simulink model "ares_single_uav_top_dirty_backup_20261011"  (R2026a)
settings: Solver=VariableStepAuto  StopTime=60
undefined symbols (not defined in the file or in its folder): DroneMass, Dx, Dy, Dz, Gravity, Ix, Iy, Iz, Lidar, MaxRange, Nx, Ny, Nz, Px, Py, Pz, UAV, Waypoints
libraries: slpidlib x6, uavsimlib x5, uavalgslib x3, robotcorelib x2
settings Model: NumberOfSteps=100  PacingRate=10  Creator=The MathWorks, Inc.  LastModifiedBy=athar
settings DebuggingCC: ParameterPrecisionLossMsg=none

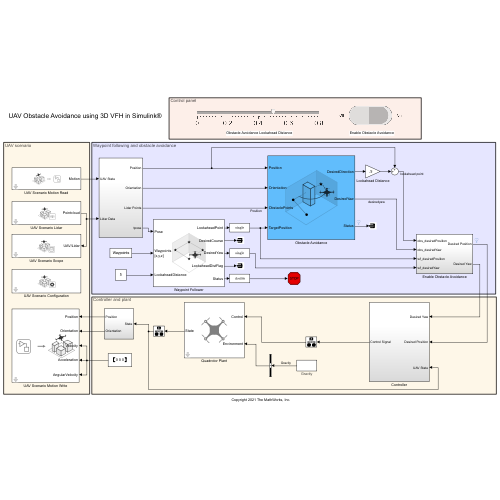
[thumbnail: Simulink's stored preview of the top-level diagram]
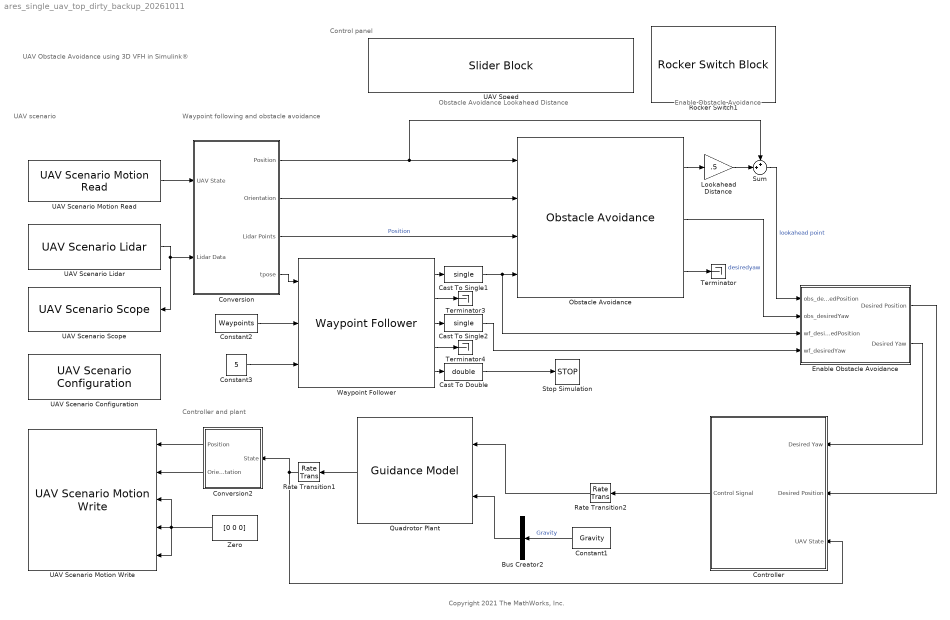
== system ares_single_uav_top_dirty_backup_20261011 ==
  note: Copyright 2021 The MathWorks, Inc.
  note: Control panel
  note: Enable Obstacle Avoidance
  note: Obstacle Avoidance Lookahead Distance
  note: Waypoint following and obstacle avoidance
  note: UAV scenario
  note: Controller and plant
  note: UAV Obstacle Avoidance using 3D VFH in Simulink®
  Bus Creator2 : BusCreator  Inputs=1  OutDataTypeStr=Bus: uavGuidanceEnvironmentBus  NonVirtualBus=on
  Cast To Double : DataTypeConversion  OutDataTypeStr=double  SaturateOnIntegerOverflow=off  RndMeth=Floor
  Cast To Single1 : DataTypeConversion  OutDataTypeStr=single  SaturateOnIntegerOverflow=off  RndMeth=Floor
  Cast To Single2 : DataTypeConversion  OutDataTypeStr=single  SaturateOnIntegerOverflow=off  RndMeth=Floor
  Constant1 : Constant  Value=Gravity  OutDataTypeStr=single
      settings: AttributesFormatString=%<Value>
  Constant2 : Constant  Value=Waypoints
  Constant3 : Constant  Value=5
  Controller : Subsystem
  Conversion : Subsystem
  Conversion2 : Subsystem
  Enable Obstacle Avoidance : Subsystem
  Lookahead Distance : Gain  Gain=.5
  Obstacle Avoidance : uavalgslib/Obstacle Avoidance  DistanceLimits=[ 0.2, MaxRange]  HorizontalSensorFOV=AzimuthLimits  VerticalSensorFOV=ElevationLimits  SensorLocation=[ 0, 0, -0.4]  SensorOrientation=[ 180, 0, 0 ]  VehicleRadius=VehicleRadius  SafetyDistance=AvoidanceSafetyDistance  SimulateUsing=Interpreted execution  HistRes=6  WindowSize=1  HistogramThreshold=1  MaxAge=3  TargetDirectionWeight=5  CurrentDirectionWeight=2  PreviousDirectionWeight=2
  Quadrotor Plant : uavalgslib/Guidance Model  ModelType=MultirotorGuidance  NumInstances=1  SpecifiedDataType=single  SimulateUsing=Code generation  InitialWorldPositionMultirotor=InitialPosition'  InitialWorldVelocityMultirotor=[0; 0; 0]  InitialEulerZYXMultirotor=|  InitialBodyAngularRateRPYMultirotor=[0; 0; 0]  InitialThrustMultirotor=0  InitialNorthFixedWing=0  InitialEastFixedWing=0  InitialHeightFixedWing=0  InitialAirSpeedFixedWing=0  InitialHeadingAngleFixedWing=0  InitialFlightPathAngleFixedWing=0  InitialRollAngleFixedWing=0  InitialRollAngleRateFixedWing=0  PDRollMultirotor=[3402.97,116.67]  PDPitchMultirotor=[3402.97, 116.67]  PYawRateMultirotor=1950  PThrustMultirotor=3900  MassMultirotor=0.1  PHeightFixedWing=3.9  PHeadingAngleFixedWing=3.9  PFlightPathAngleFixedWing=39  PDRollFixedWing=[3402.97, 116.67]  PAirSpeedFixedWing=1  FlightPathAngleLimitsFixedWing=[-pi/2, pi/2]  StateBusName='uavGuidanceStateBus'  ControlBusName='uavGuidanceControlBus'  EnvironmentBusName='uavGuidanceEnvironmentBus'  DataType=single
      | [ 0
      | ;0;0]
      link override EnvironmentSignalSpecification: OutDataTypeStr=Bus: MultirotorGuidanceEnvironmentBus
  Rate Transition1 : RateTransition  OutPortSampleTime=UAVSampleTime
  Rate Transition2 : RateTransition  OutPortSampleTime=UAVSampleTime
  Rocker Switch1 : RockerSwitchBlock  LabelPosition=Hide
  Stop Simulation : Stop
  Sum : Sum  Inputs=++|
  Terminator : Terminator
  Terminator3 : Terminator
  Terminator4 : Terminator
  UAV Scenario Configuration : uavsimlib/UAV Scenario Configuration  Priority=-1  UAVScenarioObject=Scenario  SampleTime=0.1  UpdateParam=true  SensorMotionBusName='SensorMotionBus'  PlatformMotionBusName='PlatformMotionBus'  ScenarioMotionBusName='ScenarioMotionBus'  ScenarioMotionSignalName='ScenarioMotions'
  UAV Scenario Lidar : uavsimlib/UAV Scenario Lidar  Priority=1  SensorName=UAV/Lidar  MaxRange=MaxRange  RangeAccuracy=0.02  AzimuthLimits=AzimuthLimits  AzimuthResolution=AzimuthResolution  ElevationLimits=ElevationLimits  ElevationResolution=ElevationResolution  HasNoise=off  HasOrganizedOutput=on  SampleTime=0.1
  UAV Scenario Motion Read : uavsimlib/UAV Scenario Motion Read  Priority=1  EntityName='UAV'  ReferenceFrame=NED  OutputWind=off
  UAV Scenario Motion Write : uavsimlib/UAV Scenario Motion Write  Priority=0  PlatName='UAV'  ReferenceFrame=NED
  UAV Scenario Scope : uavsimlib/UAV Scenario Scope  Priority=1  SensorNameTable={ 'UAV/Lidar', 'on' }  SampleTime=.1
  UAV Speed : SliderBlock  LabelPosition=Hide  ScaleMin=0.0  ScaleMax=.8  TickInterval=.2
  Waypoint Follower : uavalgslib/Waypoint Follower  UAVType=multirotor  StartFrom=first  TransitionRadiusSource=internal  TransitionRadius=.1  MinLookaheadDistance=.2  HoverAtLastWaypoint=off  InterpolateYaw=on  YawInput=off  ShowCrossTrackErrorOutput=off  ShowStatusOutput=on  ShowWaypointIndexOutput=off  SimulateUsing=Code generation
  Zero : Constant  Value=[0 0 0]  OutDataTypeStr=Inherit: Inherit via back propagation
  wires:
  Controller/1(Control Signal) -> Rate Transition2/1
  Rate Transition2/1 -> Quadrotor Plant/1
  Obstacle Avoidance/1 -> Lookahead Distance/1
  Rate Transition1/1 -> Controller/3(UAV State), Conversion2/1(State)
  Quadrotor Plant/1 -> Rate Transition1/1
  Conversion/1(Position) -> Sum/1, Obstacle Avoidance/1
  Conversion/2(Orientation) -> Obstacle Avoidance/2
  Bus Creator2/1 -> Quadrotor Plant/2
  Constant1/1 -> Bus Creator2/1  "Gravity"
  Lookahead Distance/1 -> Sum/2
  Obstacle Avoidance/3 -> Terminator/1
  Conversion/3(Lidar Points) -> Obstacle Avoidance/3  "Position"
  UAV Scenario Motion Read/1 -> Conversion/1(UAV State)
  UAV Scenario Lidar/1 -> UAV Scenario Scope/1, Conversion/2(Lidar Data)
  Conversion2/1(Position) -> UAV Scenario Motion Write/1
  Conversion2/2(Orientation) -> UAV Scenario Motion Write/2
  Zero/1 -> UAV Scenario Motion Write/3, UAV Scenario Motion Write/4, UAV Scenario Motion Write/5
  Waypoint Follower/5 -> Cast To Double/1
  Waypoint Follower/4 -> Terminator4/1
  Waypoint Follower/2 -> Terminator3/1
  Constant3/1 -> Waypoint Follower/3
  Waypoint Follower/1 -> Cast To Single1/1
  Constant2/1 -> Waypoint Follower/2
  Conversion/4(tpose) -> Waypoint Follower/1
  Cast To Single1/1 -> Enable Obstacle Avoidance/3(wf_desiredPosition), Obstacle Avoidance/4
  Cast To Double/1 -> Stop Simulation/1
  Waypoint Follower/3 -> Cast To Single2/1
  Sum/1 -> Enable Obstacle Avoidance/1(obs_desiredPosition)  "lookahead point"
  Obstacle Avoidance/2 -> Enable Obstacle Avoidance/2(obs_desiredYaw)  "desiredyaw"
  Cast To Single2/1 -> Enable Obstacle Avoidance/4(wf_desiredYaw)
  Enable Obstacle Avoidance/2(Desired Yaw) -> Controller/1(Desired Yaw)
  Enable Obstacle Avoidance/1(Desired Position) -> Controller/2(Desired Position)

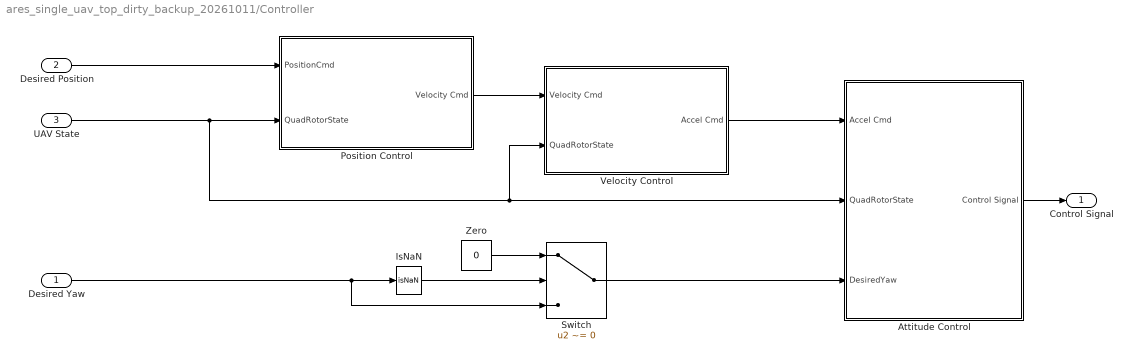
== system ares_single_uav_top_dirty_backup_20261011/Controller ==
  Desired Yaw : Inport
  Desired Position : Inport  Port=2
  UAV State : Inport  Port=3
  Attitude Control : Subsystem
  IsNaN : RelationalOperator  Operator=isNaN  OutDataTypeStr=boolean  RndMeth=Simplest  InputSameDT=off
  Position Control : Subsystem
  Switch : Switch  Criteria=u2 ~= 0  SaturateOnIntegerOverflow=off  InputSameDT=off
  Velocity Control : Subsystem
  Zero : Constant  Value=0  OutDataTypeStr=Inherit: Inherit via back propagation
  Control Signal : Outport
  wires:
  Desired Position/1 -> Position Control/1(PositionCmd)
  Velocity Control/1(Accel Cmd) -> Attitude Control/1(Accel Cmd)
  Attitude Control/1(Control Signal) -> Control Signal/1
  UAV State/1 -> Position Control/2(QuadRotorState), Velocity Control/2(QuadRotorState), Attitude Control/2(QuadRotorState)
  Position Control/1(Velocity Cmd) -> Velocity Control/1(Velocity Cmd)
  Zero/1 -> Switch/1
  IsNaN/1 -> Switch/2
  Desired Yaw/1 -> Switch/3, IsNaN/1
  Switch/1 -> Attitude Control/3(DesiredYaw)

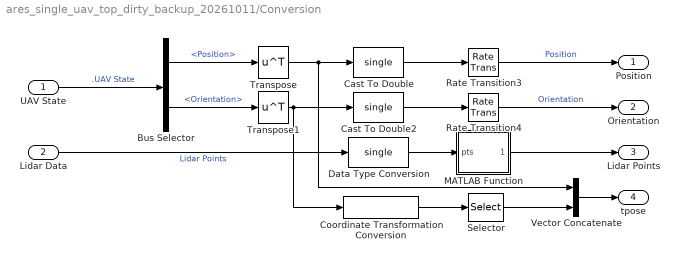
== system ares_single_uav_top_dirty_backup_20261011/Conversion ==
  UAV State : Inport
  Lidar Data : Inport  Port=2
  Bus Selector : BusSelector  OutputSignals=Position,Orientation
  Cast To Double : DataTypeConversion  OutDataTypeStr=single  SaturateOnIntegerOverflow=off  RndMeth=Floor
  Cast To Double2 : DataTypeConversion  OutDataTypeStr=single  SaturateOnIntegerOverflow=off  RndMeth=Floor
  Coordinate Transformation Conversion : robotcorelib/Coordinate Transformation Conversion  InputRepresentation=Quaternion  InputEulerSequence=ZYX  ShowTrVecInputPort=on  OutputRepresentation=Euler Angles  OutputEulerSequence=ZYX  ShowTrVecOutputPort=on  SimulateUsing=Interpreted execution
  Data Type Conversion : DataTypeConversion  OutDataTypeStr=single  SaturateOnIntegerOverflow=off  RndMeth=Floor
  MATLAB Function : MATLAB Function  TreatAsAtomicUnit=on
  Rate Transition3 : RateTransition  OutPortSampleTime=.1
  Rate Transition4 : RateTransition  OutPortSampleTime=0.1
  Selector : Selector  InputPortWidth=3  IndexOptions=Index vector (dialog)  Indices=[1]  OutputSizes=1
  Transpose : Math  Operator=transpose
  Transpose1 : Math  Operator=transpose
  Vector Concatenate : Concatenate
  Position : Outport
  Orientation : Outport  Port=2
  Lidar Points : Outport  Port=3
  tpose : Outport  Port=4
  wires:
  Bus Selector/2 -> Transpose1/1  "<Orientation>"
  Data Type Conversion/1 -> MATLAB Function/1(pts)
  Bus Selector/1 -> Transpose/1  "<Position>"
  Transpose1/1 -> Coordinate Transformation Conversion/1, Cast To Double2/1
  Transpose/1 -> Cast To Double/1, Vector Concatenate/1
  Cast To Double2/1 -> Rate Transition4/1
  UAV State/1 -> Bus Selector/1  ".UAV State"
  Lidar Data/1 -> Data Type Conversion/1  "Lidar Points"
  Rate Transition4/1 -> Orientation/1  "Orientation"
  MATLAB Function/1(points) -> Lidar Points/1
  Rate Transition3/1 -> Position/1  "Position"
  Vector Concatenate/1 -> tpose/1
  Selector/1 -> Vector Concatenate/2
  Cast To Double/1 -> Rate Transition3/1
  Coordinate Transformation Conversion/1 -> Selector/1

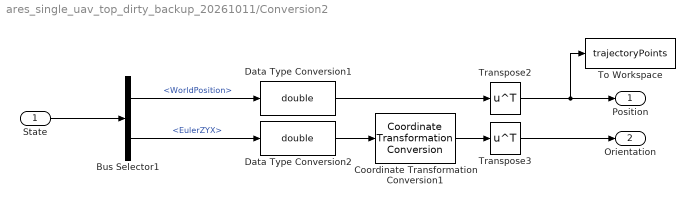
== system ares_single_uav_top_dirty_backup_20261011/Conversion2 ==
  State : Inport
  Bus Selector1 : BusSelector  OutputSignals=WorldPosition,EulerZYX
  Coordinate Transformation Conversion1 : robotcorelib/Coordinate Transformation Conversion  InputRepresentation=Euler Angles  InputEulerSequence=ZYX  ShowTrVecInputPort=on  OutputRepresentation=Quaternion  OutputEulerSequence=ZYX  ShowTrVecOutputPort=on  SimulateUsing=Code generation
  Data Type Conversion1 : DataTypeConversion  OutDataTypeStr=double  SaturateOnIntegerOverflow=off  RndMeth=Floor
  Data Type Conversion2 : DataTypeConversion  OutDataTypeStr=double  SaturateOnIntegerOverflow=off  RndMeth=Floor
  To Workspace : ToWorkspace  VariableName=trajectoryPoints  SampleTime=-1
  Transpose2 : Math  Operator=transpose
  Transpose3 : Math  Operator=transpose
  Position : Outport
  Orientation : Outport  Port=2
  wires:
  State/1 -> Bus Selector1/1
  Transpose2/1 -> To Workspace/1, Position/1
  Bus Selector1/1 -> Data Type Conversion1/1  "<WorldPosition>"
  Data Type Conversion2/1 -> Coordinate Transformation Conversion1/1
  Bus Selector1/2 -> Data Type Conversion2/1  "<EulerZYX>"
  Coordinate Transformation Conversion1/1 -> Transpose3/1
  Transpose3/1 -> Orientation/1
  Data Type Conversion1/1 -> Transpose2/1

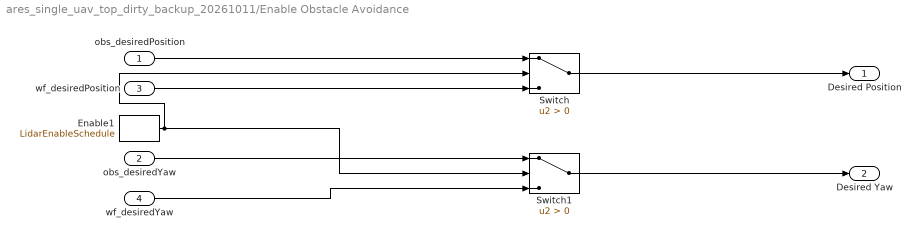
== system ares_single_uav_top_dirty_backup_20261011/Enable Obstacle Avoidance ==
  obs_desiredPosition : Inport
  obs_desiredYaw : Inport  Port=2
  wf_desiredPosition : Inport  Port=3
  wf_desiredYaw : Inport  Port=4
  Enable1 : FromWorkspace  VariableName=LidarEnableSchedule  Interpolate=off  OutputAfterFinalValue=Holding final value
  Switch : Switch  Criteria=u2 > Threshold  SaturateOnIntegerOverflow=off  InputSameDT=off
  Switch1 : Switch  Criteria=u2 > Threshold  SaturateOnIntegerOverflow=off  InputSameDT=off
  Desired Position : Outport
  Desired Yaw : Outport  Port=2
  wires:
  wf_desiredYaw/1 -> Switch1/3
  obs_desiredYaw/1 -> Switch1/1
  Switch/1 -> Desired Position/1
  obs_desiredPosition/1 -> Switch/1
  Switch1/1 -> Desired Yaw/1
  wf_desiredPosition/1 -> Switch/3
  Enable1/1 -> Switch/2, Switch1/2

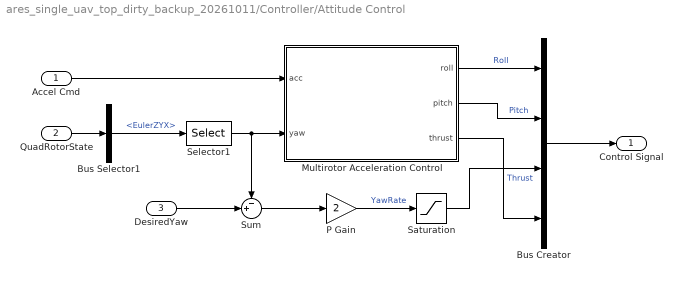
== system ares_single_uav_top_dirty_backup_20261011/Controller/Attitude Control ==
  Accel Cmd : Inport
  QuadRotorState : Inport  Port=2
  DesiredYaw : Inport  Port=3
  Bus Creator : BusCreator  Inputs=4  OutDataTypeStr=Bus: uavGuidanceControlBus  NonVirtualBus=on
      settings: InheritFromInputs=off
  Bus Selector1 : BusSelector  OutputSignals=EulerZYX
  Multirotor Acceleration Control : MATLAB Function  TreatAsAtomicUnit=on
  P Gain : Gain  Gain=2
  Saturation : Saturate
  Selector1 : Selector  InputPortWidth=3  IndexOptions=Index vector (dialog)  Indices=[1]  OutputSizes=1
  Sum : Sum  Inputs=-+|
  Control Signal : Outport
  wires:
  Selector1/1 -> Multirotor Acceleration Control/2(yaw), Sum/1
  Bus Creator/1 -> Control Signal/1
  Sum/1 -> P Gain/1
  Multirotor Acceleration Control/1(roll) -> Bus Creator/1  "Roll"
  Multirotor Acceleration Control/2(pitch) -> Bus Creator/2  "Pitch"
  Multirotor Acceleration Control/3(thrust) -> Bus Creator/4  "Thrust"
  P Gain/1 -> Saturation/1  "YawRate"
  Accel Cmd/1 -> Multirotor Acceleration Control/1(acc)
  QuadRotorState/1 -> Bus Selector1/1
  Bus Selector1/1 -> Selector1/1  "<EulerZYX>"
  Saturation/1 -> Bus Creator/3
  DesiredYaw/1 -> Sum/2

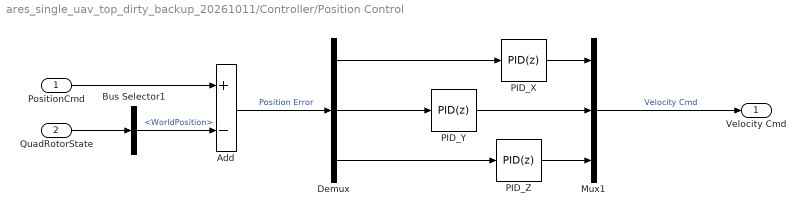
== system ares_single_uav_top_dirty_backup_20261011/Controller/Position Control ==
  PositionCmd : Inport
  QuadRotorState : Inport  Port=2
  Add : Sum  Inputs=+-
  Bus Selector1 : BusSelector  OutputSignals=WorldPosition
  Demux : Demux  Outputs=3
  Mux1 : Mux  Inputs=3
  PID_X : slpidlib/PID Controller  Controller=PID  Form=Parallel  TimeDomain=Discrete-time  UseExternalTs=off  SampleTime=-1  IntegratorMethod=Forward Euler  FilterMethod=Forward Euler  ControllerParametersSource=internal  P=Px  I=Ix  UseKiTs=off  D=Dx  UseExternalDerivativeSource=off  N=Nx  UseFilter=on  TunerSelectOption=Transfer Function Based (PID Tuner App)  InitialConditionSource=internal  InitialConditionForIntegrator=0  InitialConditionForFilter=0  DifferentiatorICPrevScaledInput=0  ExternalReset=none  TrackingMode=off  Kt=1  LimitOutput=on  SatLimitsSource=internal  UpperSaturationLimit=3  LowerSaturationLimit=-3  LinearizeAsGain=on  AntiWindupMode=clamping  Kb=1  LimitIntegrator=off  UpperIntegratorSaturationLimit=inf  LowerIntegratorSaturationLimit=-inf  POutMin=[]  POutMax=[]  IOutMin=[]  IOutMax=[]  DOutMin=[]  DOutMax=[]  NOutMin=[]  NOutMax=[]  SumOutMin=[]  SumOutMax=[]  SaturationOutMin=[]  SaturationOutMax=[]  PParamMin=[]  PParamMax=[]  IParamMin=[]  IParamMax=[]  DParamMin=[]  DParamMax=[]  NParamMin=[]  NParamMax=[]  KbParamMin=[]  KbParamMax=[]  KtParamMin=[]  KtParamMax=[]  KbOutMin=[]  KbOutMax=[]  KtOutMin=[]  KtOutMax=[]  IntegratorOutMin=[]  IntegratorOutMax=[]  FilterOutMin=[]  FilterOutMax=[]  SumI1OutMin=SumI1OutMin  SumI1OutMax=SumI1OutMax  SumI2OutMin=[]  SumI2OutMax=[]  SumI3OutMin=[]  SumI3OutMax=[]  SumI4OutMin=[]  SumI4OutMax=[]  SumDOutMin=[]  SumDOutMax=[]  DifferentiatorOutMin=[]  DifferentiatorOutMax=[]  FilterDiffOutCoefMin=[]  FilterDiffOutCoefMax=[]  ReciprocalOutMin=[]  ReciprocalOutMax=[]  SumDenOutMin=[]  SumDenOutMax=[]  SumNumOutMin=[]  SumNumOutMax=[]  DivideOutMin=[]  DivideOutMax=[]  UdiffTsProdOutMin=[]  UdiffTsProdOutMax=[]  NTsProdOutMin=[]  NTsProdOutMax=[]  UintegralTsProdOutMin=[]  UintegralTsProdOutMax=[]  UngainTsProdOutMin=[]  UngainTsProdOutMax=[]  ClampingZeroOutDataTypeStr=Inherit: Inherit via back propagation  ClampingZeroOutMin=[]  ClampingZeroOutMax=[]  FilterDenConstantOutDataTypeStr=Inherit: Inherit via back propagation  FilterDenConstantOutMin=[]  FilterDenConstantOutMax=[]  PCopyOutDataTypeStr=Inherit: Inherit via back propagation  PCopyOutMin=[]  PCopyOutMax=[]  NCopyOutDataTypeStr=Inherit: Inherit via back propagation  NCopyOutMin=[]  NCopyOutMax=[]  IntegratorContinuousStateAttributes=''  IntegratorStateMustResolveToSignalObject=off  IntegratorRTWStateStorageClass=Auto  FilterContinuousStateAttributes=''  FilterStateMustResolveToSignalObject=off  FilterRTWStateStorageClass=Auto  ParallelPVariant=InternalParameters  IdealPVariant=Disabled  IVariant=InternalParameters  DVariant=InternalParameters  IntegratorVariant=Discrete  SatVariant=Enabled  AWVariant=DiscClampingParallel  PCopyVariant=Disabled  TRVariant=Disabled  FdbkBlocksVariant=Forward  IdealPFdbkVariant=Disabled  SatFdbkVariant=Disabled  DerivativeFilterVariant=ForwardEulerFilter  NVariant=InternalParameters  NCopyVariant=Disabled  FilterICVariant=InternalICsFilter  IntegratorICVariant=InternalICs  ExternalResetVariant=Disabled  TRSumVariant=Passthrough  SumFdbkVariant=Disabled  SumVariant=Sum_PID  TsampFilterVariant=InternalTs  TsampNgainVariant=Passthrough  TsampIntegralVariant=Disabled_SignalSpec  ExternalSaturationOutDataTypeStr=Inherit: Same as second input  DerivativeSourceVariant=ErrorSignal  PreIntVariant=InternalPreInt
      settings: AttributesFormatString=P: %<P>, I: %<I>, D:%<D>
  PID_Y : slpidlib/PID Controller  Controller=PID  Form=Parallel  TimeDomain=Discrete-time  UseExternalTs=off  SampleTime=-1  IntegratorMethod=Forward Euler  FilterMethod=Forward Euler  ControllerParametersSource=internal  P=Py  I=Iy  UseKiTs=off  D=Dy  UseExternalDerivativeSource=off  N=Ny  UseFilter=on  TunerSelectOption=Transfer Function Based (PID Tuner App)  InitialConditionSource=internal  InitialConditionForIntegrator=0  InitialConditionForFilter=0  DifferentiatorICPrevScaledInput=0  ExternalReset=none  TrackingMode=off  Kt=1  LimitOutput=on  SatLimitsSource=internal  UpperSaturationLimit=3  LowerSaturationLimit=-3  LinearizeAsGain=on  AntiWindupMode=clamping  Kb=1  LimitIntegrator=off  UpperIntegratorSaturationLimit=inf  LowerIntegratorSaturationLimit=-inf  POutMin=[]  POutMax=[]  IOutMin=[]  IOutMax=[]  DOutMin=[]  DOutMax=[]  NOutMin=[]  NOutMax=[]  SumOutMin=[]  SumOutMax=[]  SaturationOutMin=[]  SaturationOutMax=[]  PParamMin=[]  PParamMax=[]  IParamMin=[]  IParamMax=[]  DParamMin=[]  DParamMax=[]  NParamMin=[]  NParamMax=[]  KbParamMin=[]  KbParamMax=[]  KtParamMin=[]  KtParamMax=[]  KbOutMin=[]  KbOutMax=[]  KtOutMin=[]  KtOutMax=[]  IntegratorOutMin=[]  IntegratorOutMax=[]  FilterOutMin=[]  FilterOutMax=[]  SumI1OutMin=SumI1OutMin  SumI1OutMax=SumI1OutMax  SumI2OutMin=[]  SumI2OutMax=[]  SumI3OutMin=[]  SumI3OutMax=[]  SumI4OutMin=[]  SumI4OutMax=[]  SumDOutMin=[]  SumDOutMax=[]  DifferentiatorOutMin=[]  DifferentiatorOutMax=[]  FilterDiffOutCoefMin=[]  FilterDiffOutCoefMax=[]  ReciprocalOutMin=[]  ReciprocalOutMax=[]  SumDenOutMin=[]  SumDenOutMax=[]  SumNumOutMin=[]  SumNumOutMax=[]  DivideOutMin=[]  DivideOutMax=[]  UdiffTsProdOutMin=[]  UdiffTsProdOutMax=[]  NTsProdOutMin=[]  NTsProdOutMax=[]  UintegralTsProdOutMin=[]  UintegralTsProdOutMax=[]  UngainTsProdOutMin=[]  UngainTsProdOutMax=[]  ClampingZeroOutDataTypeStr=Inherit: Inherit via back propagation  ClampingZeroOutMin=[]  ClampingZeroOutMax=[]  FilterDenConstantOutDataTypeStr=Inherit: Inherit via back propagation  FilterDenConstantOutMin=[]  FilterDenConstantOutMax=[]  PCopyOutDataTypeStr=Inherit: Inherit via back propagation  PCopyOutMin=[]  PCopyOutMax=[]  NCopyOutDataTypeStr=Inherit: Inherit via back propagation  NCopyOutMin=[]  NCopyOutMax=[]  IntegratorContinuousStateAttributes=''  IntegratorStateMustResolveToSignalObject=off  IntegratorRTWStateStorageClass=Auto  FilterContinuousStateAttributes=''  FilterStateMustResolveToSignalObject=off  FilterRTWStateStorageClass=Auto  ParallelPVariant=InternalParameters  IdealPVariant=Disabled  IVariant=InternalParameters  DVariant=InternalParameters  IntegratorVariant=Discrete  SatVariant=Enabled  AWVariant=DiscClampingParallel  PCopyVariant=Disabled  TRVariant=Disabled  FdbkBlocksVariant=Forward  IdealPFdbkVariant=Disabled  SatFdbkVariant=Disabled  DerivativeFilterVariant=ForwardEulerFilter  NVariant=InternalParameters  NCopyVariant=Disabled  FilterICVariant=InternalICsFilter  IntegratorICVariant=InternalICs  ExternalResetVariant=Disabled  TRSumVariant=Passthrough  SumFdbkVariant=Disabled  SumVariant=Sum_PID  TsampFilterVariant=InternalTs  TsampNgainVariant=Passthrough  TsampIntegralVariant=Disabled_SignalSpec  ExternalSaturationOutDataTypeStr=Inherit: Same as second input  DerivativeSourceVariant=ErrorSignal  PreIntVariant=InternalPreInt
      settings: AttributesFormatString=P: %<P>, I: %<I>, D:%<D>
  PID_Z : slpidlib/PID Controller  Controller=PID  Form=Parallel  TimeDomain=Discrete-time  UseExternalTs=off  SampleTime=-1  IntegratorMethod=Forward Euler  FilterMethod=Forward Euler  ControllerParametersSource=internal  P=Pz  I=Iz  UseKiTs=off  D=Dz  UseExternalDerivativeSource=off  N=Nz  UseFilter=on  TunerSelectOption=Transfer Function Based (PID Tuner App)  InitialConditionSource=internal  InitialConditionForIntegrator=0  InitialConditionForFilter=0  DifferentiatorICPrevScaledInput=0  ExternalReset=none  TrackingMode=off  Kt=1  LimitOutput=on  SatLimitsSource=internal  UpperSaturationLimit=3  LowerSaturationLimit=-3  LinearizeAsGain=on  AntiWindupMode=clamping  Kb=1  LimitIntegrator=off  UpperIntegratorSaturationLimit=inf  LowerIntegratorSaturationLimit=-inf  POutMin=[]  POutMax=[]  IOutMin=[]  IOutMax=[]  DOutMin=[]  DOutMax=[]  NOutMin=[]  NOutMax=[]  SumOutMin=[]  SumOutMax=[]  SaturationOutMin=[]  SaturationOutMax=[]  PParamMin=[]  PParamMax=[]  IParamMin=[]  IParamMax=[]  DParamMin=[]  DParamMax=[]  NParamMin=[]  NParamMax=[]  KbParamMin=[]  KbParamMax=[]  KtParamMin=[]  KtParamMax=[]  KbOutMin=[]  KbOutMax=[]  KtOutMin=[]  KtOutMax=[]  IntegratorOutMin=[]  IntegratorOutMax=[]  FilterOutMin=[]  FilterOutMax=[]  SumI1OutMin=SumI1OutMin  SumI1OutMax=SumI1OutMax  SumI2OutMin=[]  SumI2OutMax=[]  SumI3OutMin=[]  SumI3OutMax=[]  SumI4OutMin=[]  SumI4OutMax=[]  SumDOutMin=[]  SumDOutMax=[]  DifferentiatorOutMin=[]  DifferentiatorOutMax=[]  FilterDiffOutCoefMin=[]  FilterDiffOutCoefMax=[]  ReciprocalOutMin=[]  ReciprocalOutMax=[]  SumDenOutMin=[]  SumDenOutMax=[]  SumNumOutMin=[]  SumNumOutMax=[]  DivideOutMin=[]  DivideOutMax=[]  UdiffTsProdOutMin=[]  UdiffTsProdOutMax=[]  NTsProdOutMin=[]  NTsProdOutMax=[]  UintegralTsProdOutMin=[]  UintegralTsProdOutMax=[]  UngainTsProdOutMin=[]  UngainTsProdOutMax=[]  ClampingZeroOutDataTypeStr=Inherit: Inherit via back propagation  ClampingZeroOutMin=[]  ClampingZeroOutMax=[]  FilterDenConstantOutDataTypeStr=Inherit: Inherit via back propagation  FilterDenConstantOutMin=[]  FilterDenConstantOutMax=[]  PCopyOutDataTypeStr=Inherit: Inherit via back propagation  PCopyOutMin=[]  PCopyOutMax=[]  NCopyOutDataTypeStr=Inherit: Inherit via back propagation  NCopyOutMin=[]  NCopyOutMax=[]  IntegratorContinuousStateAttributes=''  IntegratorStateMustResolveToSignalObject=off  IntegratorRTWStateStorageClass=Auto  FilterContinuousStateAttributes=''  FilterStateMustResolveToSignalObject=off  FilterRTWStateStorageClass=Auto  ParallelPVariant=InternalParameters  IdealPVariant=Disabled  IVariant=InternalParameters  DVariant=InternalParameters  IntegratorVariant=Discrete  SatVariant=Enabled  AWVariant=DiscClampingParallel  PCopyVariant=Disabled  TRVariant=Disabled  FdbkBlocksVariant=Forward  IdealPFdbkVariant=Disabled  SatFdbkVariant=Disabled  DerivativeFilterVariant=ForwardEulerFilter  NVariant=InternalParameters  NCopyVariant=Disabled  FilterICVariant=InternalICsFilter  IntegratorICVariant=InternalICs  ExternalResetVariant=Disabled  TRSumVariant=Passthrough  SumFdbkVariant=Disabled  SumVariant=Sum_PID  TsampFilterVariant=InternalTs  TsampNgainVariant=Passthrough  TsampIntegralVariant=Disabled_SignalSpec  ExternalSaturationOutDataTypeStr=Inherit: Same as second input  DerivativeSourceVariant=ErrorSignal  PreIntVariant=InternalPreInt
      settings: AttributesFormatString=P: %<P>, I: %<I>, D:%<D>
  Velocity Cmd : Outport
  wires:
  Demux/3 -> PID_Z/1
  Demux/1 -> PID_X/1
  PID_Z/1 -> Mux1/3
  Add/1 -> Demux/1  "Position Error"
  Demux/2 -> PID_Y/1
  Mux1/1 -> Velocity Cmd/1  "Velocity Cmd"
  PID_X/1 -> Mux1/1
  PID_Y/1 -> Mux1/2
  Bus Selector1/1 -> Add/2  "<WorldPosition>"
  QuadRotorState/1 -> Bus Selector1/1
  PositionCmd/1 -> Add/1

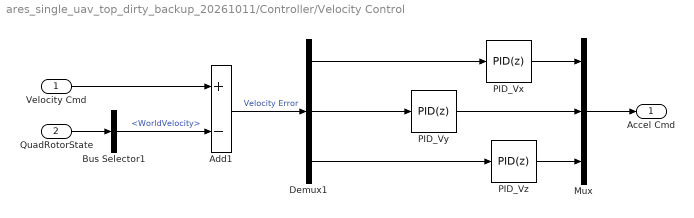
== system ares_single_uav_top_dirty_backup_20261011/Controller/Velocity Control ==
  Velocity Cmd : Inport
  QuadRotorState : Inport  Port=2
  Add1 : Sum  Inputs=+-
  Bus Selector1 : BusSelector  OutputSignals=WorldVelocity
  Demux1 : Demux  Outputs=3
  Mux : Mux  Inputs=3
  PID_Vx : slpidlib/PID Controller  Controller=PID  Form=Parallel  TimeDomain=Discrete-time  UseExternalTs=off  SampleTime=-1  IntegratorMethod=Forward Euler  FilterMethod=Forward Euler  ControllerParametersSource=internal  P=Px  I=Ix  UseKiTs=off  D=Dx  UseExternalDerivativeSource=off  N=Nx  UseFilter=on  TunerSelectOption=Transfer Function Based (PID Tuner App)  InitialConditionSource=internal  InitialConditionForIntegrator=0  InitialConditionForFilter=0  DifferentiatorICPrevScaledInput=0  ExternalReset=none  TrackingMode=off  Kt=1  LimitOutput=on  SatLimitsSource=internal  UpperSaturationLimit=1  LowerSaturationLimit=-1  LinearizeAsGain=on  AntiWindupMode=clamping  Kb=1  LimitIntegrator=off  UpperIntegratorSaturationLimit=inf  LowerIntegratorSaturationLimit=-inf  POutMin=[]  POutMax=[]  IOutMin=[]  IOutMax=[]  DOutMin=[]  DOutMax=[]  NOutMin=[]  NOutMax=[]  SumOutMin=[]  SumOutMax=[]  SaturationOutMin=[]  SaturationOutMax=[]  PParamMin=[]  PParamMax=[]  IParamMin=[]  IParamMax=[]  DParamMin=[]  DParamMax=[]  NParamMin=[]  NParamMax=[]  KbParamMin=[]  KbParamMax=[]  KtParamMin=[]  KtParamMax=[]  KbOutMin=[]  KbOutMax=[]  KtOutMin=[]  KtOutMax=[]  IntegratorOutMin=[]  IntegratorOutMax=[]  FilterOutMin=[]  FilterOutMax=[]  SumI1OutMin=SumI1OutMin  SumI1OutMax=SumI1OutMax  SumI2OutMin=[]  SumI2OutMax=[]  SumI3OutMin=[]  SumI3OutMax=[]  SumI4OutMin=[]  SumI4OutMax=[]  SumDOutMin=[]  SumDOutMax=[]  DifferentiatorOutMin=[]  DifferentiatorOutMax=[]  FilterDiffOutCoefMin=[]  FilterDiffOutCoefMax=[]  ReciprocalOutMin=[]  ReciprocalOutMax=[]  SumDenOutMin=[]  SumDenOutMax=[]  SumNumOutMin=[]  SumNumOutMax=[]  DivideOutMin=[]  DivideOutMax=[]  UdiffTsProdOutMin=[]  UdiffTsProdOutMax=[]  NTsProdOutMin=[]  NTsProdOutMax=[]  UintegralTsProdOutMin=[]  UintegralTsProdOutMax=[]  UngainTsProdOutMin=[]  UngainTsProdOutMax=[]  ClampingZeroOutDataTypeStr=Inherit: Inherit via back propagation  ClampingZeroOutMin=[]  ClampingZeroOutMax=[]  FilterDenConstantOutDataTypeStr=Inherit: Inherit via back propagation  FilterDenConstantOutMin=[]  FilterDenConstantOutMax=[]  PCopyOutDataTypeStr=Inherit: Inherit via back propagation  PCopyOutMin=[]  PCopyOutMax=[]  NCopyOutDataTypeStr=Inherit: Inherit via back propagation  NCopyOutMin=[]  NCopyOutMax=[]  IntegratorContinuousStateAttributes=''  IntegratorStateMustResolveToSignalObject=off  IntegratorRTWStateStorageClass=Auto  FilterContinuousStateAttributes=''  FilterStateMustResolveToSignalObject=off  FilterRTWStateStorageClass=Auto  ParallelPVariant=InternalParameters  IdealPVariant=Disabled  IVariant=InternalParameters  DVariant=InternalParameters  IntegratorVariant=Discrete  SatVariant=Enabled  AWVariant=DiscClampingParallel  PCopyVariant=Disabled  TRVariant=Disabled  FdbkBlocksVariant=Forward  IdealPFdbkVariant=Disabled  SatFdbkVariant=Disabled  DerivativeFilterVariant=ForwardEulerFilter  NVariant=InternalParameters  NCopyVariant=Disabled  FilterICVariant=InternalICsFilter  IntegratorICVariant=InternalICs  ExternalResetVariant=Disabled  TRSumVariant=Passthrough  SumFdbkVariant=Disabled  SumVariant=Sum_PID  TsampFilterVariant=InternalTs  TsampNgainVariant=Passthrough  TsampIntegralVariant=Disabled_SignalSpec  ExternalSaturationOutDataTypeStr=Inherit: Same as second input  DerivativeSourceVariant=ErrorSignal  PreIntVariant=InternalPreInt
      settings: AttributesFormatString=P: %<P>, I: %<I>, D:%<D>
  PID_Vy : slpidlib/PID Controller  Controller=PID  Form=Parallel  TimeDomain=Discrete-time  UseExternalTs=off  SampleTime=-1  IntegratorMethod=Forward Euler  FilterMethod=Forward Euler  ControllerParametersSource=internal  P=Py  I=Iy  UseKiTs=off  D=Dy  UseExternalDerivativeSource=off  N=Ny  UseFilter=on  TunerSelectOption=Transfer Function Based (PID Tuner App)  InitialConditionSource=internal  InitialConditionForIntegrator=0  InitialConditionForFilter=0  DifferentiatorICPrevScaledInput=0  ExternalReset=none  TrackingMode=off  Kt=1  LimitOutput=on  SatLimitsSource=internal  UpperSaturationLimit=1  LowerSaturationLimit=-1  LinearizeAsGain=on  AntiWindupMode=clamping  Kb=1  LimitIntegrator=off  UpperIntegratorSaturationLimit=inf  LowerIntegratorSaturationLimit=-inf  POutMin=[]  POutMax=[]  IOutMin=[]  IOutMax=[]  DOutMin=[]  DOutMax=[]  NOutMin=[]  NOutMax=[]  SumOutMin=[]  SumOutMax=[]  SaturationOutMin=[]  SaturationOutMax=[]  PParamMin=[]  PParamMax=[]  IParamMin=[]  IParamMax=[]  DParamMin=[]  DParamMax=[]  NParamMin=[]  NParamMax=[]  KbParamMin=[]  KbParamMax=[]  KtParamMin=[]  KtParamMax=[]  KbOutMin=[]  KbOutMax=[]  KtOutMin=[]  KtOutMax=[]  IntegratorOutMin=[]  IntegratorOutMax=[]  FilterOutMin=[]  FilterOutMax=[]  SumI1OutMin=SumI1OutMin  SumI1OutMax=SumI1OutMax  SumI2OutMin=[]  SumI2OutMax=[]  SumI3OutMin=[]  SumI3OutMax=[]  SumI4OutMin=[]  SumI4OutMax=[]  SumDOutMin=[]  SumDOutMax=[]  DifferentiatorOutMin=[]  DifferentiatorOutMax=[]  FilterDiffOutCoefMin=[]  FilterDiffOutCoefMax=[]  ReciprocalOutMin=[]  ReciprocalOutMax=[]  SumDenOutMin=[]  SumDenOutMax=[]  SumNumOutMin=[]  SumNumOutMax=[]  DivideOutMin=[]  DivideOutMax=[]  UdiffTsProdOutMin=[]  UdiffTsProdOutMax=[]  NTsProdOutMin=[]  NTsProdOutMax=[]  UintegralTsProdOutMin=[]  UintegralTsProdOutMax=[]  UngainTsProdOutMin=[]  UngainTsProdOutMax=[]  ClampingZeroOutDataTypeStr=Inherit: Inherit via back propagation  ClampingZeroOutMin=[]  ClampingZeroOutMax=[]  FilterDenConstantOutDataTypeStr=Inherit: Inherit via back propagation  FilterDenConstantOutMin=[]  FilterDenConstantOutMax=[]  PCopyOutDataTypeStr=Inherit: Inherit via back propagation  PCopyOutMin=[]  PCopyOutMax=[]  NCopyOutDataTypeStr=Inherit: Inherit via back propagation  NCopyOutMin=[]  NCopyOutMax=[]  IntegratorContinuousStateAttributes=''  IntegratorStateMustResolveToSignalObject=off  IntegratorRTWStateStorageClass=Auto  FilterContinuousStateAttributes=''  FilterStateMustResolveToSignalObject=off  FilterRTWStateStorageClass=Auto  ParallelPVariant=InternalParameters  IdealPVariant=Disabled  IVariant=InternalParameters  DVariant=InternalParameters  IntegratorVariant=Discrete  SatVariant=Enabled  AWVariant=DiscClampingParallel  PCopyVariant=Disabled  TRVariant=Disabled  FdbkBlocksVariant=Forward  IdealPFdbkVariant=Disabled  SatFdbkVariant=Disabled  DerivativeFilterVariant=ForwardEulerFilter  NVariant=InternalParameters  NCopyVariant=Disabled  FilterICVariant=InternalICsFilter  IntegratorICVariant=InternalICs  ExternalResetVariant=Disabled  TRSumVariant=Passthrough  SumFdbkVariant=Disabled  SumVariant=Sum_PID  TsampFilterVariant=InternalTs  TsampNgainVariant=Passthrough  TsampIntegralVariant=Disabled_SignalSpec  ExternalSaturationOutDataTypeStr=Inherit: Same as second input  DerivativeSourceVariant=ErrorSignal  PreIntVariant=InternalPreInt
      settings: AttributesFormatString=P: %<P>, I: %<I>, D:%<D>
  PID_Vz : slpidlib/PID Controller  Controller=PID  Form=Parallel  TimeDomain=Discrete-time  UseExternalTs=off  SampleTime=-1  IntegratorMethod=Forward Euler  FilterMethod=Forward Euler  ControllerParametersSource=internal  P=Pz  I=Iz  UseKiTs=off  D=Dz  UseExternalDerivativeSource=off  N=Nz  UseFilter=on  TunerSelectOption=Transfer Function Based (PID Tuner App)  InitialConditionSource=internal  InitialConditionForIntegrator=0  InitialConditionForFilter=0  DifferentiatorICPrevScaledInput=0  ExternalReset=none  TrackingMode=off  Kt=1  LimitOutput=on  SatLimitsSource=internal  UpperSaturationLimit=4  LowerSaturationLimit=-4  LinearizeAsGain=on  AntiWindupMode=clamping  Kb=1  LimitIntegrator=off  UpperIntegratorSaturationLimit=inf  LowerIntegratorSaturationLimit=-inf  POutMin=[]  POutMax=[]  IOutMin=[]  IOutMax=[]  DOutMin=[]  DOutMax=[]  NOutMin=[]  NOutMax=[]  SumOutMin=[]  SumOutMax=[]  SaturationOutMin=[]  SaturationOutMax=[]  PParamMin=[]  PParamMax=[]  IParamMin=[]  IParamMax=[]  DParamMin=[]  DParamMax=[]  NParamMin=[]  NParamMax=[]  KbParamMin=[]  KbParamMax=[]  KtParamMin=[]  KtParamMax=[]  KbOutMin=[]  KbOutMax=[]  KtOutMin=[]  KtOutMax=[]  IntegratorOutMin=[]  IntegratorOutMax=[]  FilterOutMin=[]  FilterOutMax=[]  SumI1OutMin=SumI1OutMin  SumI1OutMax=SumI1OutMax  SumI2OutMin=[]  SumI2OutMax=[]  SumI3OutMin=[]  SumI3OutMax=[]  SumI4OutMin=[]  SumI4OutMax=[]  SumDOutMin=[]  SumDOutMax=[]  DifferentiatorOutMin=[]  DifferentiatorOutMax=[]  FilterDiffOutCoefMin=[]  FilterDiffOutCoefMax=[]  ReciprocalOutMin=[]  ReciprocalOutMax=[]  SumDenOutMin=[]  SumDenOutMax=[]  SumNumOutMin=[]  SumNumOutMax=[]  DivideOutMin=[]  DivideOutMax=[]  UdiffTsProdOutMin=[]  UdiffTsProdOutMax=[]  NTsProdOutMin=[]  NTsProdOutMax=[]  UintegralTsProdOutMin=[]  UintegralTsProdOutMax=[]  UngainTsProdOutMin=[]  UngainTsProdOutMax=[]  ClampingZeroOutDataTypeStr=Inherit: Inherit via back propagation  ClampingZeroOutMin=[]  ClampingZeroOutMax=[]  FilterDenConstantOutDataTypeStr=Inherit: Inherit via back propagation  FilterDenConstantOutMin=[]  FilterDenConstantOutMax=[]  PCopyOutDataTypeStr=Inherit: Inherit via back propagation  PCopyOutMin=[]  PCopyOutMax=[]  NCopyOutDataTypeStr=Inherit: Inherit via back propagation  NCopyOutMin=[]  NCopyOutMax=[]  IntegratorContinuousStateAttributes=''  IntegratorStateMustResolveToSignalObject=off  IntegratorRTWStateStorageClass=Auto  FilterContinuousStateAttributes=''  FilterStateMustResolveToSignalObject=off  FilterRTWStateStorageClass=Auto  ParallelPVariant=InternalParameters  IdealPVariant=Disabled  IVariant=InternalParameters  DVariant=InternalParameters  IntegratorVariant=Discrete  SatVariant=Enabled  AWVariant=DiscClampingParallel  PCopyVariant=Disabled  TRVariant=Disabled  FdbkBlocksVariant=Forward  IdealPFdbkVariant=Disabled  SatFdbkVariant=Disabled  DerivativeFilterVariant=ForwardEulerFilter  NVariant=InternalParameters  NCopyVariant=Disabled  FilterICVariant=InternalICsFilter  IntegratorICVariant=InternalICs  ExternalResetVariant=Disabled  TRSumVariant=Passthrough  SumFdbkVariant=Disabled  SumVariant=Sum_PID  TsampFilterVariant=InternalTs  TsampNgainVariant=Passthrough  TsampIntegralVariant=Disabled_SignalSpec  ExternalSaturationOutDataTypeStr=Inherit: Same as second input  DerivativeSourceVariant=ErrorSignal  PreIntVariant=InternalPreInt
      settings: AttributesFormatString=P: %<P>, I: %<I>, D:%<D>
  Accel Cmd : Outport
  wires:
  Add1/1 -> Demux1/1  "Velocity Error"
  PID_Vz/1 -> Mux/3
  Demux1/1 -> PID_Vx/1
  PID_Vy/1 -> Mux/2
  Velocity Cmd/1 -> Add1/1
  Demux1/3 -> PID_Vz/1
  Mux/1 -> Accel Cmd/1
  PID_Vx/1 -> Mux/1
  Demux1/2 -> PID_Vy/1
  Bus Selector1/1 -> Add1/2  "<WorldVelocity>"
  QuadRotorState/1 -> Bus Selector1/1

== matlab function ares_single_uav_top_dirty_backup_20261011/Conversion/MATLAB Function ==
  data: pts input; points output
function points = lidarToPoints(pts)

xLidar = reshape(pts(:,:,1),[],1);
yLidar = reshape(pts(:,:,2),[],1);
zLidar = reshape(pts(:,:,3),[],1);
    
points = [xLidar,yLidar,zLidar];

== matlab function ares_single_uav_top_dirty_backup_20261011/Controller/Attitude Control/Multirotor Acceleration Control ==
  data: acc input; roll output; pitch output; thrust output; yaw input; DroneMass parameter; Gravity parameter
function [roll, pitch, thrust] = accControl(acc, yaw, DroneMass, Gravity)

    xddot = acc(1);
    yddot = acc(2);
    zddot = acc(3);
    
    pitch = atan2((-xddot*cos(yaw)-yddot*sin(yaw)), ( -zddot + Gravity));
    roll = atan2(((-xddot*sin(yaw)+yddot*cos(yaw))*cos(pitch)), (-zddot+Gravity));
    
    roll_limit = 25*pi/180;
    pitch_limit = 25*pi/180;
    
    roll = min(roll_limit, max(-roll_limit, roll));
   
    pitch = min(pitch_limit, max(-pitch_limit, pitch));
    
    thrust = DroneMass*(-zddot+Gravity)/(cos(pitch)*cos(roll));
end
